simulink model "dc_motor_open_loop"  (R2024b)
settings: Solver=FixedStepAuto  StartTime=0.0  StopTime=10.0  FixedStep=0.01  RelTol=1e-3
undefined symbols (not defined in the file or in its folder): motor, p
settings Model: Creator=Taha  LastModifiedBy=Taha
settings OptimizationCC: DefaultParameterBehavior=Inlined  UseDivisionForNetSlopeComputation=on  GainParamInheritBuiltInType=on  UseFloatMulNetSlope=on  InlineInvariantSignals=on  PassReuseOutputArgsAs=Individual arguments  ZeroExternalMemoryAtStartup=off  ZeroInternalMemoryAtStartup=off  NoFixptDivByZeroProtection=on  EfficientFloat2IntCast=on  LifeSpan=1  OptimizeBlockOrder=speed  DifferentSizesBufferReuse=on  EfficientTunableParamExpr=on
settings DebuggingCC: ParameterTunabilityLossMsg=error
settings HardwareCC: ProdLongLongMode=on
settings SFSimCC: MATLABDynamicMemAlloc=off
settings RTWCC: Description=Embedded Coder  SystemTargetFile=ert.tlc  TemplateMakefile=ert_default_tmf
settings CodeAppCC: ForceParamTrailComments=on  IgnoreCustomStorageClasses=off  OperatorAnnotations=on  SimulinkDataObjDesc=on  SFDataObjDesc=on  CustomSymbolStrGlobalVar=rt$N$M  CustomSymbolStrType=$N$M  CustomSymbolStrFcn=$N$M$F  CustomSymbolStrMacro=$N$M  InsertBlockDesc=on
settings ERTTargetCC: TargetLangStandard=C99 (ISO)  GenerateSampleERTMain=on  IncludeMdlTerminateFcn=off  CombineSignalStateStructs=on  SupportComplex=off  SupportContinuousTime=on  ERTCustomFileTemplate=example_file_process.tlc  ERTFilePackagingFormat=CompactWithDataFile

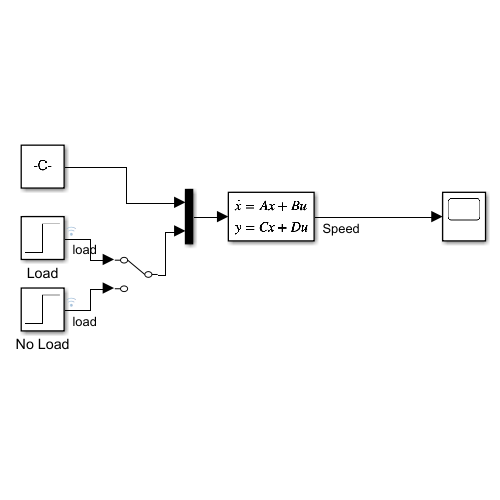
[thumbnail: Simulink's stored preview of the top-level diagram]
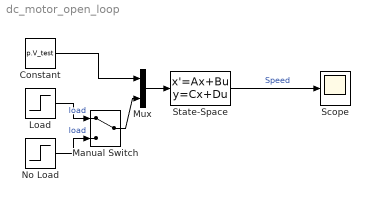
== system dc_motor_open_loop ==
  Constant : Constant  Value=p.V_test
  Load : Step  Time=p.t_load  After=p.TL_test  SampleTime=0
  Manual Switch : ManualSwitch
  Mux : Mux  Inputs=2
  No Load : Step  Time=p.t_load  After=0  SampleTime=0
  Scope : Scope
  State-Space : StateSpace  A=motor.A  B=motor.B  C=motor.C  D=motor.D  InitialCondition=0
  wires:
  Constant/1 -> Mux/1
  State-Space/1 -> Scope/1  "Speed"
  Mux/1 -> State-Space/1
  Manual Switch/1 -> Mux/2
  No Load/1 -> Manual Switch/2  "load"
  Load/1 -> Manual Switch/1  "load"
